simulink model "PWM_Rectifier_30V"  (R2021b)
settings: Solver=FixedStepAuto  StartTime=0.0  StopTime=1  RelTol=1e-3
libraries: spsSeriesRLCBranchLib x3, spsMeanLib x3, spsVoltageMeasurementLib x3, spsACVoltageSourceLib x1, spsCurrentMeasurementLib x1, powerlib_extras x1, spsParallelRLCBranchLib x1, spsTHDLib x1, spsUniversalBridgeLib x1, spspowerguiLib x1, simulink x1, slpidlib x1
settings Model: Creator=abc6820292  LastModifiedBy=abc6820292
settings SolverCC: ZeroCrossControl=EnableAll  ZeroCrossAlgorithm=Adaptive
settings DataIOCC: ReturnWorkspaceOutputs=off  Refine=10
settings DebuggingCC: IgnoredZcDiagnostic=none

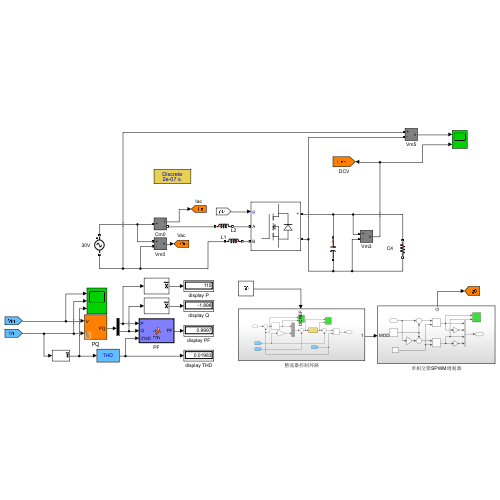
[thumbnail: Simulink's stored preview of the top-level diagram]
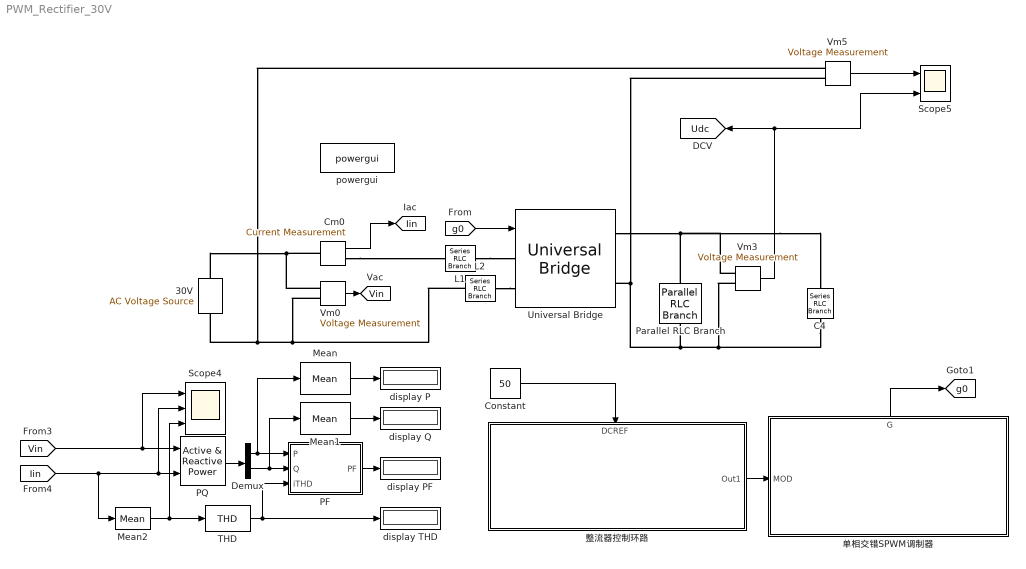
== system PWM_Rectifier_30V ==
  30V : spsACVoltageSourceLib/AC Voltage Source  Amplitude=42  Phase=0  Frequency=50  SampleTime=0  Measurements=None  BusType=swing  Pref=10e3  Qref=0  Qmin=-inf  Qmax=+inf
  C4 : spsSeriesRLCBranchLib/Series RLC Branch  LConnTagsString=__new0  RConnTagsString=__new0  BranchType=R  Resistance=20  Inductance=0.1  SetiL0=off  InitialCurrent=0  Capacitance=2e-3  Setx0=on  InitialVoltage=350  Measurements=None
  Cm0 : spsCurrentMeasurementLib/Current Measurement  PhasorSimulation=off  OutputType=Complex  PSBequivalent=0
  Constant : Constant  Value=50
  Demux : Demux  Outputs=2
  L1 : spsSeriesRLCBranchLib/Series RLC Branch  LConnTagsString=__new0  RConnTagsString=__new0  BranchType=L  Resistance=2000  Inductance=4.7e-4  SetiL0=off  InitialCurrent=0  Capacitance=2e-3  Setx0=on  InitialVoltage=350  Measurements=None
  L2 : spsSeriesRLCBranchLib/Series RLC Branch  LConnTagsString=__new0  RConnTagsString=__new0  BranchType=L  Resistance=2000  Inductance=4.7e-4  SetiL0=off  InitialCurrent=0  Capacitance=2e-3  Setx0=on  InitialVoltage=350  Measurements=None
  Mean : spsMeanLib/Mean  Freq=50  Vinit=0  Ts=0
  Mean1 : spsMeanLib/Mean  Freq=50  Vinit=0  Ts=0
  Mean2 : spsMeanLib/Mean  Freq=2000  Vinit=0  Ts=0
  PF : MATLAB Function  TreatAsAtomicUnit=on
  PQ : powerlib_extras/Measurements/Active & Reactive Power  f1=60
      settings: SourceProductBaseCode=PS
  Parallel RLC Branch : spsParallelRLCBranchLib/Parallel RLC Branch  LConnTagsString=a  RConnTagsString=__new0  BranchType=C  Resistance=1e3  Inductance=1e-3  SetiL0=off  InitialCurrent=0  Capacitance=6e-3  Setx0=on  InitialVoltage=42  Measurements=None
  Scope4 : Scope  NumInputPorts=3
  Scope5 : Scope  NumInputPorts=2
  THD : spsTHDLib/THD  Freq=50  Ts=0
      settings: SourceProductBaseCode=PS
  Universal Bridge : spsUniversalBridgeLib/Universal Bridge  Arms=2  SnubberResistance=1e5  SnubberCapacitance=inf  Device=MOSFET / Diodes  Ron=1e-3  Lon=0  ForwardVoltages="[  0  0  ]"  ForwardVoltage=0  GTOparameters=[ 10e-6 , 20e-6 ]  IGBTparameters=[ 1e-6 , 2e-6 ]  Measurements=None  Measurements_2=None  converterType=Rectifier
  Vm0 : spsVoltageMeasurementLib/Voltage Measurement  PhasorSimulation=off  OutputType=Complex  PSBequivalent=0
  Vm3 : spsVoltageMeasurementLib/Voltage Measurement  PhasorSimulation=off  OutputType=Complex  PSBequivalent=0
  Vm5 : spsVoltageMeasurementLib/Voltage Measurement  PhasorSimulation=off  OutputType=Complex  PSBequivalent=0
  display P : Display
  display PF : Display
  display Q : Display
  display THD : Display
  powergui : spspowerguiLib/powergui  SimulationMode=Discrete  SampleTime=2e-7  frequency=60  Iterations=50  frequencyindice=0  Pbase=100e6  ErrMax=1e-4  UnitsV=kV  UnitsW=MW  buscounter=0  FunctionMessages=off  echomessages=off  EnableUseOfTLC=off  CurrentSourceSwitches=off  DisableSnubberDevices=off  DisableRonSwitches=off  DisableVfSwitches=off  DisplayEquations=off  AutomaticDiscreteSolvers=off  SolverType=Tustin/Backward Euler (TBE)  Interpol=off  ExternalGateDelay=off  methode=off  Ts=0  x0status=blocks  SPID=off  SwTol=0  HookPort=off  NonlinearTolerance=1e-4  nMaxIteration=100  ContinueOnMaxIteration=off  RestoreLinks=warning  ResistiveCurrentMeasurement=off  Frange=[0:2:500]  Ylog=off  Xlog=on  ShowGrid=off  save=off  variable=ZData  structure=QQQQQ  ZoomFFT=off  StartTime=0.5  cycles=15  DisplayStyle=1  fundamental=50  FreqAxis=off  MaxFrequency=1000  frequencyindicesteady=1  RmsSteady=1  display=off
  单相交错SPWM调制器 : Subsystem
      settings: PortSchema="{\"entries\":[{\"content\":{\"sides\":[{\"content\":{\"connectorIds\":[\"In1\"]},\"type\":\"ConnectorPlacement.EquallySpacedRectSide\",\"uuid\":\"d8d9f1c1-8f81-406f-b923-78e82289e6f2\"},{\"content\":{\"connectorIds\":[],\"side\":\"RIGHT\"},\"type\":\"ConnectorPlacement.EquallySpacedRectSide\",\"uuid\":\"2d6088a2-038d-47a3-8186-5a9123353715\"},{\"content\":{\"connectorIds\":[\"Out1\"],\"side\":\"TOP\"},\"type\":\"ConnectorPlacement.EquallySpacedRectSide\",\"uuid\":\"23c9a0a4-4c71-40c7-bbf8-b7d214677c68\"}]},\"type\":\"ConnectorPlacement.EquallySpacedConnector\",\"uuid\":\"f578564d-2c11-4354-b186-026709011600\"}],\"packageUris\":[\"http://schema.mathworks.com/mf0/Connector/R2020b\"],\"version\":\"1.0\"}"
  整流器控制环路 : Subsystem
      settings: PortSchema="{\"entries\":[{\"content\":{\"sides\":[{\"content\":{\"connectorIds\":[]},\"type\":\"ConnectorPlacement.EquallySpacedRectSide\",\"uuid\":\"884483d4-93ce-45a0-b2f2-f4a386f6ac62\"},{\"content\":{\"connectorIds\":[\"Out1\"],\"side\":\"RIGHT\"},\"type\":\"ConnectorPlacement.EquallySpacedRectSide\",\"uuid\":\"6f7c7192-aa4b-45c6-a8d7-02f9fc8abf55\"},{\"content\":{\"connectorIds\":[\"In1\"],\"side\":\"TOP\"},\"type\":\"ConnectorPlacement.EquallySpacedRectSide\",\"uuid\":\"a90d3442-663c-4783-b290-5421ca40f1c7\"}]},\"type\":\"ConnectorPlacement.EquallySpacedConnector\",\"uuid\":\"49045a45-1409-4b85-a90b-3b97b614be91\"}],\"packageUris\":[\"http://schema.mathworks.com/mf0/Connector/R2020b\"],\"version\":\"1.0\"}"
  tag scope: Iin=global, Udc=global, Vin=global, g0=global
  wires:
  Vm3/1 -> [Udc], Scope5/2
  Vm0/1 -> [Vin]
  [Vin] -> Scope4/1, PQ/1
  PQ/1 -> Demux/1
  Demux/1 -> Mean/1, PF/1(P)
  Demux/2 -> Mean1/1, PF/2(Q)
  THD/1 -> display THD/1, PF/3(iTHD)
  PF/1(PF) -> display PF/1
  Mean/1 -> display P/1
  Mean1/1 -> display Q/1
  [g0] -> Universal Bridge/1
  单相交错SPWM调制器/1(G) -> [g0]
  Cm0/1 -> [Iin]
  [Iin] -> Mean2/1, Scope4/2, PQ/2
  整流器控制环路/1(Out1) -> 单相交错SPWM调制器/1(MOD)
  Mean2/1 -> Scope4/3, THD/1
  Vm5/1 -> Scope5/1
  Constant/1 -> 整流器控制环路/1(DCREF)
  connections:
  C4/RConn1 -- Vm5/LConn2 -- Universal Bridge/RConn2 -- Parallel RLC Branch/RConn1 -- Vm3/LConn2
  Cm0/LConn1 -- Vm0/LConn1 -- 30V/RConn1
  Vm0/LConn2 -- L2/RConn1 -- 30V/LConn1 -- Vm5/LConn1
  Parallel RLC Branch/LConn1 -- Universal Bridge/RConn1 -- Vm3/LConn1 -- C4/LConn1
  L1/RConn1 -- Universal Bridge/LConn1
  L2/LConn1 -- Universal Bridge/LConn2
  Cm0/RConn1 -- L1/LConn1

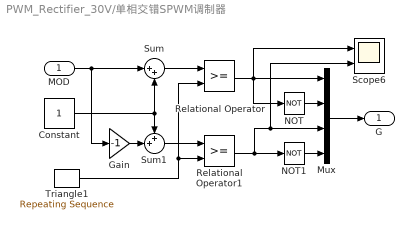
== system PWM_Rectifier_30V/单相交错SPWM调制器 ==
  MOD : Inport
  Constant : Constant
  Gain : Gain  Gain=-1
  Mux : Mux
  NOT : Logic  Operator=NOT  IconShape=distinctive  AllPortsSameDT=off  OutDataTypeStr=boolean
  NOT1 : Logic  Operator=NOT  IconShape=distinctive  AllPortsSameDT=off  OutDataTypeStr=boolean
  Relational Operator : RelationalOperator  OutDataTypeStr=boolean  RndMeth=Nearest
  Relational Operator1 : RelationalOperator  OutDataTypeStr=boolean  RndMeth=Nearest
  Scope6 : Scope  NumInputPorts=2
  Sum : Sum  Inputs=|++
  Sum1 : Sum  Inputs=++|
  Triangle1 : simulink/Sources/Repeating Sequence  rep_seq_t=[0 1/20000/2 1/20000]  rep_seq_y=[0 2 0]
  G : Outport
  wires:
  Triangle1/1 -> Relational Operator1/2, Relational Operator/2
  Mux/1 -> G/1
  NOT/1 -> Mux/2
  Relational Operator/1 -> Scope6/1, Mux/1, NOT/1
  MOD/1 -> Sum/1, Gain/1
  Sum/1 -> Relational Operator/1
  Sum1/1 -> Relational Operator1/1
  Relational Operator1/1 -> Scope6/2, Mux/3, NOT1/1
  Constant/1 -> Sum1/1, Sum/2
  Gain/1 -> Sum1/2
  NOT1/1 -> Mux/4

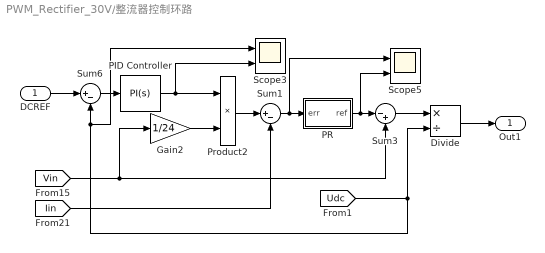
== system PWM_Rectifier_30V/整流器控制环路 ==
  DCREF : Inport
  Divide : Product  Inputs=*/
  Gain2 : Gain  Gain=1/24
  PID Controller : slpidlib/PID Controller  Controller=PI  Form=Parallel  TimeDomain=Continuous-time  UseExternalTs=off  SampleTime=-1  IntegratorMethod=Forward Euler  FilterMethod=Forward Euler  ControllerParametersSource=internal  P=0.1  I=5  D=0.005  UseFilter=on  N=100  TunerSelectOption=Transfer Function Based (PID Tuner App)  InitialConditionSource=internal  InitialConditionForIntegrator=0  InitialConditionForFilter=0  DifferentiatorICPrevScaledInput=0  ExternalReset=none  TrackingMode=off  Kt=1  LimitOutput=on  SatLimitsSource=internal  UpperSaturationLimit=100  LowerSaturationLimit=-20  LinearizeAsGain=on  AntiWindupMode=clamping  Kb=1  POutMin=[]  POutMax=[]  IOutMin=[]  IOutMax=[]  DOutMin=[]  DOutMax=[]  NOutMin=[]  NOutMax=[]  SumOutMin=[]  SumOutMax=[]  SaturationOutMin=[]  SaturationOutMax=[]  PParamMin=[]  PParamMax=[]  IParamMin=[]  IParamMax=[]  DParamMin=[]  DParamMax=[]  NParamMin=[]  NParamMax=[]  KbParamMin=[]  KbParamMax=[]  KtParamMin=[]  KtParamMax=[]  KbOutMin=[]  KbOutMax=[]  KtOutMin=[]  KtOutMax=[]  IntegratorOutMin=[]  IntegratorOutMax=[]  FilterOutMin=[]  FilterOutMax=[]  SumI1OutMin=[]  SumI1OutMax=[]  SumI2OutMin=[]  SumI2OutMax=[]  SumI3OutMin=[]  SumI3OutMax=[]  SumI4OutMin=[]  SumI4OutMax=[]  SumDOutMin=[]  SumDOutMax=[]  DifferentiatorOutMin=[]  DifferentiatorOutMax=[]  FilterDiffOutCoefMin=[]  FilterDiffOutCoefMax=[]  ReciprocalOutMin=[]  ReciprocalOutMax=[]  SumDenOutMin=[]  SumDenOutMax=[]  SumNumOutMin=[]  SumNumOutMax=[]  DivideOutMin=[]  DivideOutMax=[]  UdiffTsProdOutMin=[]  UdiffTsProdOutMax=[]  NTsProdOutMin=[]  NTsProdOutMax=[]  UintegralTsProdOutMin=[]  UintegralTsProdOutMax=[]  UngainTsProdOutMin=[]  UngainTsProdOutMax=[]  FilterDenConstantOutDataTypeStr=Inherit: Inherit via back propagation  FilterDenConstantOutMin=[]  FilterDenConstantOutMax=[]  PCopyOutDataTypeStr=Inherit: Inherit via back propagation  PCopyOutMin=[]  PCopyOutMax=[]  NCopyOutDataTypeStr=Inherit: Inherit via back propagation  NCopyOutMin=[]  NCopyOutMax=[]  IntegratorContinuousStateAttributes=''  IntegratorStateMustResolveToSignalObject=off  IntegratorRTWStateStorageClass=Auto  FilterContinuousStateAttributes=''  FilterStateMustResolveToSignalObject=off  FilterRTWStateStorageClass=Auto  ParallelPVariant=InternalParameters  IdealPVariant=Disabled  IVariant=InternalParameters  DVariant=Disabled  IntegratorVariant=Continuous  SatVariant=Enabled  AWVariant=ContClampingParallel  PCopyVariant=Disabled  TRVariant=Disabled  FdbkBlocksVariant=Forward  IdealPFdbkVariant=Disabled  SatFdbkVariant=Disabled  DerivativeFilterVariant=Disabled  NVariant=Disabled  NCopyVariant=Disabled_SignalSpec  FilterICVariant=Disabled  IntegratorICVariant=InternalICs  ExternalResetVariant=Disabled  TRSumVariant=Passthrough  SumFdbkVariant=Disabled  SumVariant=Sum_PI  TsampFilterVariant=InternalTs  TsampNgainVariant=Passthrough  TsampIntegralVariant=Passthrough  ExternalSaturationOutDataTypeStr=Inherit: Same as second input
  PR : Subsystem  TreatAsAtomicUnit=on  mask{Kp=8, Kr=100, Wc=5, Upper=1200, Lower=-1200}
  Product2 : Product  RndMeth=Zero
  Scope3 : Scope  NumInputPorts=2
  Scope5 : Scope  NumInputPorts=2
  Sum1 : Sum  Inputs=|+-
  Sum3 : Sum  Inputs=|-+
  Sum6 : Sum  Inputs=|+-
  Out1 : Outport
  wires:
  Divide/1 -> Out1/1
  Sum6/1 -> PID Controller/1
  [Vin] -> Sum3/2, Gain2/1
  PR/1(ref) -> Sum3/1, Scope5/2
  [Iin] -> Sum1/2
  Sum3/1 -> Divide/1
  Sum1/1 -> Scope5/1, PR/1(err)
  PID Controller/1 -> Product2/1, Scope3/2
  Product2/1 -> Sum1/1
  Gain2/1 -> Product2/2
  DCREF/1 -> Sum6/1
  [Udc] -> Scope3/1, Sum6/2, Divide/2

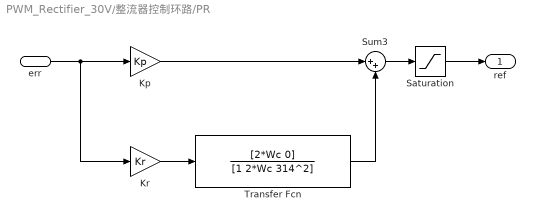
== system PWM_Rectifier_30V/整流器控制环路/PR ==
  err : Inport
  Kp : Gain  Gain=Kp
  Kr : Gain  Gain=Kr
  Saturation : Saturate  UpperLimit=Upper  LowerLimit=Lower
  Sum3 : Sum  Inputs=|++
  Transfer Fcn : TransferFcn  Numerator=[2*Wc 0]  Denominator=[1 2*Wc 314^2]
  ref : Outport
  wires:
  Kp/1 -> Sum3/1
  Sum3/1 -> Saturation/1
  err/1 -> Kr/1, Kp/1
  Kr/1 -> Transfer Fcn/1
  Transfer Fcn/1 -> Sum3/2
  Saturation/1 -> ref/1

== matlab function PWM_Rectifier_30V/PF ==
  data: P input; PF output; Q input; iTHD input
function PF = fcn(P,Q,iTHD)
% This block supports an embeddable subset of the MATLAB language.
% See the help menu for details. 
PF=(P/sqrt(P*P+Q*Q))/(sqrt(1+iTHD*iTHD));
